simulink model "FSI01_01"  (R2024b)
settings: Solver=FixedStepAuto  StartTime=0.0  StopTime=10.0  FixedStep=0.001  RelTol=1e-3
settings Model: Creator=fmiro  LastModifiedBy=fmiro

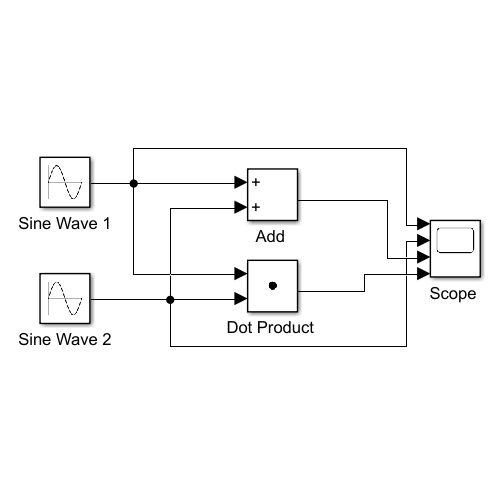
[thumbnail: Simulink's stored preview of the top-level diagram]
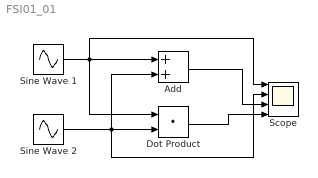
== system FSI01_01 ==
  "Add " : Sum
  "Dot Product " : DotProduct  OutDataTypeStr=Inherit: Inherit via internal rule
  "Scope " : Scope  NumInputPorts=4
  Sine Wave 1 : Sin  Amplitude=2  Frequency=3  Phase=pi  SampleTime=0
  Sine Wave 2 : Sin  SampleTime=0
  wires:
  Sine Wave 1/1 -> "Add "/1, "Scope "/1, "Dot Product "/1
  Sine Wave 2/1 -> "Dot Product "/2, "Scope "/2, "Add "/2
  "Dot Product "/1 -> "Scope "/4
  "Add "/1 -> "Scope "/3
